simulink model "control_logic"  (R2025b)
settings: Solver=VariableStepAuto  StartTime=0.0  StopTime=10.0  RelTol=1e-3
settings Model: Creator=op  LastModifiedBy=op

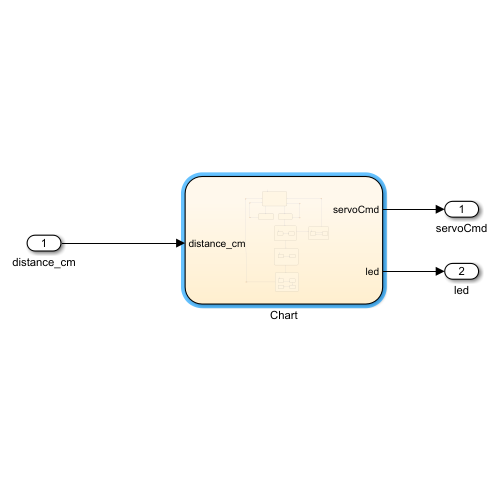
[thumbnail: Simulink's stored preview of the top-level diagram]
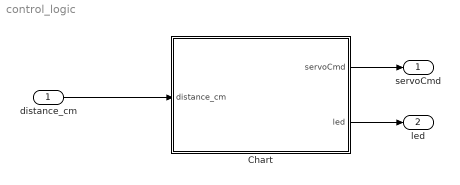
== system control_logic ==
  distance_cm : Inport
  Chart : Stateflow chart  TreatAsAtomicUnit=on
  servoCmd : Outport
  led : Outport  Port=2
  wires:
  distance_cm/1 -> Chart/1(distance_cm)
  Chart/1(servoCmd) -> servoCmd/1
  Chart/2(led) -> led/1

== stateflow chart control_logic/Chart ==
  state S_CLOSED
    entry:
    servoCmd=0;
    led=0;
  state S_VERY_CLOSE
    entry:
    servoCmd=0;
    led=1;
  state S_REQ_DET
    entry:
    servoCmd=0;
    led=0;
  state S_HALF_OPEN
    entry:
    servoCmd=90;
    state LED_ON
      entry:
      led=1;
    state LED_OFF
      entry:
      led=0;
    (default) -> S_HALF_OPEN.LED_ON
    S_HALF_OPEN.LED_ON -> S_HALF_OPEN.LED_OFF : after(1,sec)
  state S_TIMEOUT
    entry:
    servoCmd=0;
    state LED_ON
      entry:
      led=1;
    state LED_OFF
      entry:
      led=0;
    (default) -> S_TIMEOUT.LED_ON
    S_TIMEOUT.LED_ON -> S_TIMEOUT.LED_OFF : after(1,sec)
    S_TIMEOUT.LED_OFF -> S_TIMEOUT.LED_ON : after(1,sec)
  state S_OPEN
    entry:
    servoCmd=180;
    state LED_ON
      entry:
      led=1;
    state LED_OFF
      entry:
      led=0;
    (default) -> S_OPEN.LED_ON
    S_OPEN.LED_ON -> S_OPEN.LED_OFF : after(1,sec)
  state S_RESET
    entry:
    servoCmd=0;
    led=0;
    state LED_ON1
      entry:
      led=1;
    state LED_OFF1
      entry:
      led=0;
    state LED_OFF2
      entry:
      led=0;
    state LED_ON2
      entry:
      led=1;
    (default) -> LED_ON1
    LED_ON1 -> LED_OFF1 : after(1,sec)
    LED_OFF1 -> LED_ON2 : after(1,sec)
    LED_ON2 -> LED_OFF2 : after(1,sec)
  (default) -> S_CLOSED
  (junction 76) -> S_CLOSED
  (junction 17) -> S_CLOSED
  S_TIMEOUT -> (junction 76) : [distance_cm>2.5]
  (junction 14) -> (junction 17) : after(30,sec)
  (junction 28) -> S_CLOSED : [distance_cm>0.5]
  (junction 26) -> (junction 28)
  (junction 41) -> S_CLOSED
  (junction 39) -> (junction 41) : [distance_cm>2.5]
  S_CLOSED -> S_VERY_CLOSE [order 2] : [distance_cm<=0.5]
  S_CLOSED -> S_REQ_DET [order 1] : [distance_cm>0.5 && distance_cm<=2.5]
  S_VERY_CLOSE -> (junction 26)
  S_REQ_DET -> (junction 39) [order 1]
  S_REQ_DET -> S_HALF_OPEN [order 2] : [duration(distance_cm > 0.5 && distance_cm <= 2.5)>=5]
  S_HALF_OPEN -> S_TIMEOUT [order 1] : [ distance_cm>1 && after(10,sec)]
  S_HALF_OPEN -> S_OPEN [order 2] : [before(10,sec) && distance_cm <=1]
  S_OPEN -> S_RESET : after(10,sec)
  S_RESET -> (junction 14)
  data: distance_cm input; servoCmd output; led output
